simulink model "Simulacion_PIL_Ideal"  (R2026a)
settings: Solver=VariableStepAuto  StopTime=2000  FixedStep=0.05  MaxStep=0.001
values from neighbouring files (symbols this model uses):
  den_s0 = G1 * G_eq    (= 0.172451295072)    [Modelado.m]
  den_s1 = (C_eq * G1) + (Cp * G1) + (Cp * G_eq)    (= 95.0203777143)    [Modelado.m]
  den_s2 = C_eq * Cp    (= 11224.6716568)    [Modelado.m]
  G1 = h1 * A1    (= 0.0428065366612)    [Modelado.m]
libraries: sl_discontinuities x1
settings Model: Creator=magui  LastModifiedBy=Mariano M

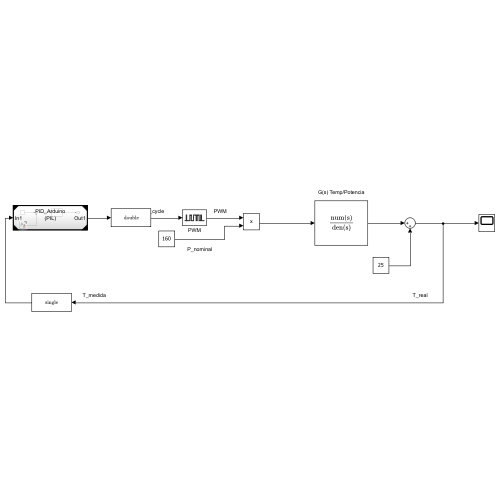
[thumbnail: Simulink's stored preview of the top-level diagram]
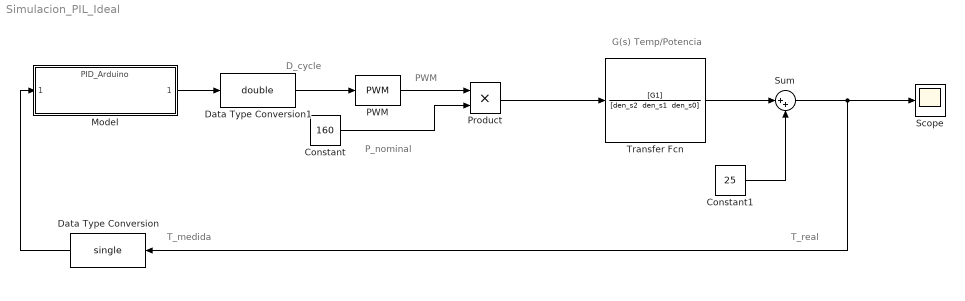
== system Simulacion_PIL_Ideal ==
  note: D_cycle
  note: T_real
  note: T_medida
  note: PWM
  note: P_nominal
  note: G(s) Temp/Potencia
  Constant : Constant  Value=160
  Constant1 : Constant  Value=25
  Data Type Conversion : DataTypeConversion  OutDataTypeStr=single  SaturateOnIntegerOverflow=off  RndMeth=Floor
  Data Type Conversion1 : DataTypeConversion  OutDataTypeStr=double  SaturateOnIntegerOverflow=off  RndMeth=Floor
  Model : ModelReference  ModelNameDialog=PID_Arduino.slx  SimulationMode=Processor-in-the-loop (PIL)  ModelReferenceVersion=1.15
  PWM : sl_discontinuities/PWM  DisableCoverage=on  Period=1/980  InitialDelay=0  DisallowZeroDutyCycle=off  RunAtFixedTimeIntervals=off  SampleTime=5e-5
      settings: LibrarySourceBlock=simulink/Discontinuities/PWM
  Product : Product
  Scope : Scope
      settings: ActiveDisplayYMinimum=4.2368956493146008  ActiveDisplayYMaximum=48.84971092344324
  Sum : Sum  Inputs=|++
  Transfer Fcn : TransferFcn  Numerator=[G1]  Denominator="[den_s2  den_s1  den_s0]"
  wires:
  Product/1 -> Transfer Fcn/1
  Constant/1 -> Product/2
  Model/1 -> Data Type Conversion1/1
  Data Type Conversion/1 -> Model/1
  Data Type Conversion1/1 -> PWM/1
  PWM/1 -> Product/1
  Transfer Fcn/1 -> Sum/1
  Sum/1 -> Data Type Conversion/1, Scope/1
  Constant1/1 -> Sum/2
